simulink model "scheme_L2"  (R2023b)
settings: Solver=ode45  StartTime=0.0  StopTime=8  MaxStep=0.001  RelTol=1e-10  AbsTol=1e-12
model workspace (MAT data in the model file):
  input_kind = 1
  pulse_width = 0.01
  sine_frequency = 1
settings Model: Creator=ASUS  LastModifiedBy=ASUS
settings DataIOCC: SaveOutput=off  SignalLogging=off  SaveTime=off

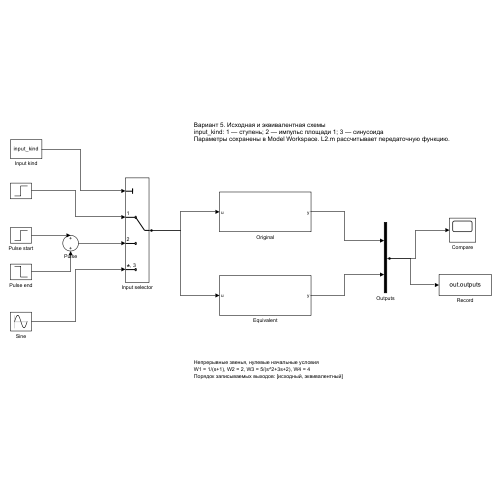
[thumbnail: Simulink's stored preview of the top-level diagram]
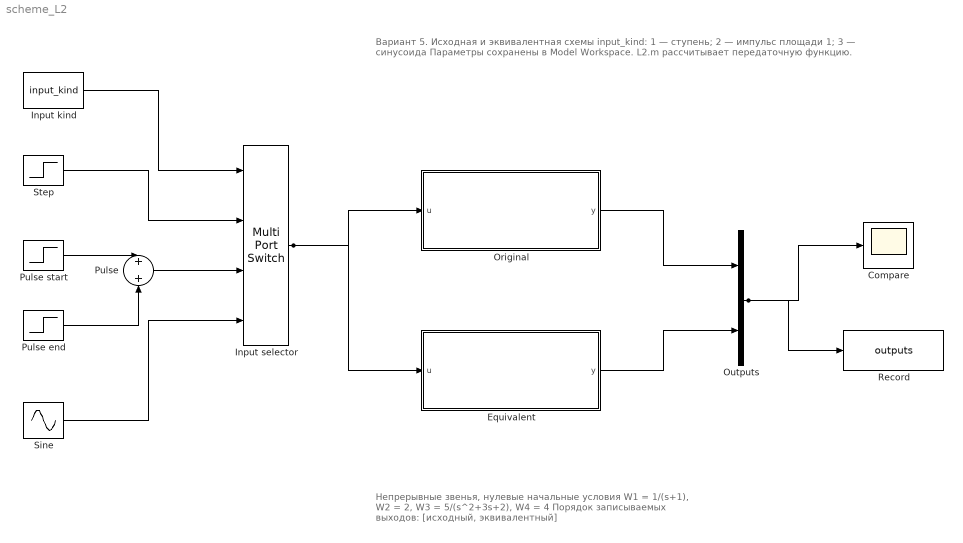
== system scheme_L2 ==
  note: Вариант 5. Исходная и эквивалентная схемы
      | input_kind: 1 — ступень; 2 — импульс площади 1; 3 — синусоида
      | Параметры сохранены в Model Workspace. L2.m рассчитывает передаточную функцию.
  note: Непрерывные звенья, нулевые начальные условия
      | W1 = 1/(s+1), W2 = 2, W3 = 5/(s^2+3s+2), W4 = 4
      | Порядок записываемых выходов: [исходный, эквивалентный]
  Compare : Scope
  Equivalent : Subsystem
  Input kind : Constant  Value=input_kind
  Input selector : MultiPortSwitch  SaturateOnIntegerOverflow=off  InputSameDT=off
  Original : Subsystem
  Outputs : Mux  Inputs=2
  Pulse : Sum
  Pulse end : Step  Time=pulse_width  After=-1/pulse_width  SampleTime=0
  Pulse start : Step  Time=0  After=1/pulse_width  SampleTime=0
  Record : ToWorkspace  VariableName=outputs  SaveFormat=Timeseries  SampleTime=-1
  Sine : Sin  Frequency=sine_frequency  SampleTime=0
  Step : Step  Time=0  SampleTime=0
  wires:
  Input kind/1 -> Input selector/1
  Step/1 -> Input selector/2
  Pulse start/1 -> Pulse/1
  Pulse end/1 -> Pulse/2
  Pulse/1 -> Input selector/3
  Sine/1 -> Input selector/4
  Input selector/1 -> Original/1(u), Equivalent/1(u)
  Original/1(y) -> Outputs/1
  Equivalent/1(y) -> Outputs/2
  Outputs/1 -> Compare/1, Record/1

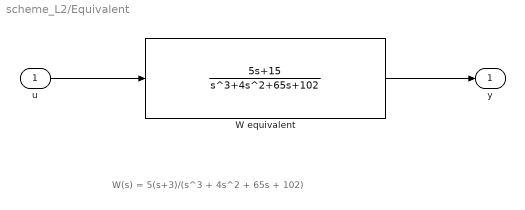
== system scheme_L2/Equivalent ==
  note: W(s) = 5(s+3)/(s^3 + 4s^2 + 65s + 102)
  u : Inport
  W equivalent : TransferFcn  Numerator=[5 15]  Denominator=[1 4 65 102]
  y : Outport
  wires:
  u/1 -> W equivalent/1
  W equivalent/1 -> y/1

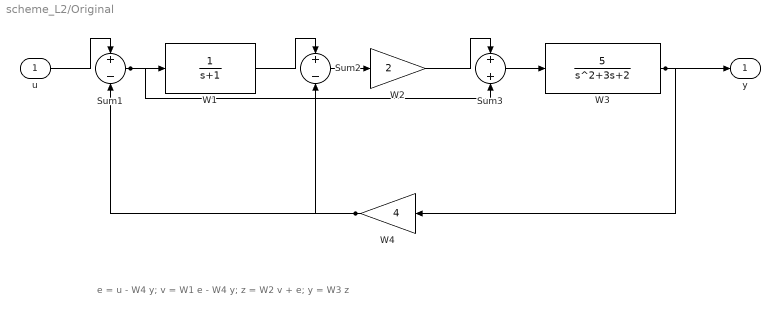
== system scheme_L2/Original ==
  note: e = u - W4 y; v = W1 e - W4 y; z = W2 v + e; y = W3 z
  u : Inport
  Sum1 : Sum  Inputs=+-
  Sum2 : Sum  Inputs=+-
  Sum3 : Sum
  W1 : TransferFcn  Denominator=[1 1]
  W2 : Gain  Gain=2
  W3 : TransferFcn  Numerator=[5]  Denominator=[1 3 2]
  W4 : Gain  Gain=4
  y : Outport
  wires:
  u/1 -> Sum1/1
  Sum1/1 -> W1/1, Sum3/2
  W1/1 -> Sum2/1
  Sum2/1 -> W2/1
  W2/1 -> Sum3/1
  Sum3/1 -> W3/1
  W3/1 -> y/1, W4/1
  W4/1 -> Sum1/2, Sum2/2
